simulink subsystem "Main_Controller_Scopes"  (R2025a)
settings: Solver=VariableStepAuto  StartTime=0.0  StopTime=10.0  RelTol=1e-3
Description:
  | Copyright 2025 The MathWorks, Inc.
settings Model: Creator=smiller  LastModifiedBy=smiller

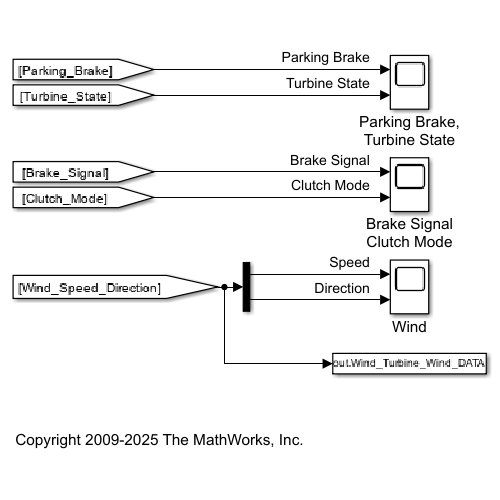
[thumbnail: Simulink's stored preview of the top-level diagram]
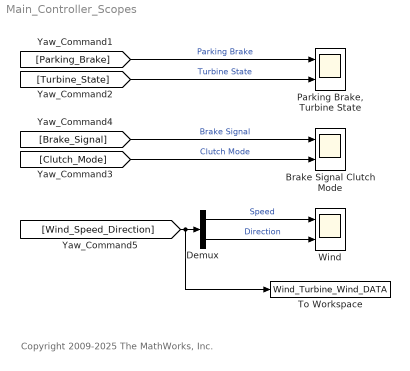
== system Main_Controller_Scopes ==
  note: Copyright 2009-2025 The MathWorks, Inc.
  Brake Signal Clutch Mode : Scope  NumInputPorts=2
      settings: TimeSpan=80  ActiveDisplayYMinimum=-1  ActiveDisplayYMaximum=1
  Demux : Demux  Outputs=2
  "Parking Brake, Turbine State" : Scope  NumInputPorts=2
      settings: TimeSpan=80  ActiveDisplayYMinimum=0  ActiveDisplayYMaximum=1  DataLoggingVariableName=ScopeData2
  To Workspace : ToWorkspace  VariableName=Wind_Turbine_Wind_DATA  SaveFormat=Structure With Time  SampleTime=-1
  Wind : Scope  NumInputPorts=2
      settings: TimeSpan=80  ActiveDisplayYMinimum=0  ActiveDisplayYMaximum=20  DataLoggingVariableName=Wind_Turbine_Wind_DATA
  wires:
  Demux/2 -> Wind/2  "Direction"
  [Clutch_Mode] -> Brake Signal Clutch Mode/2  "Clutch Mode"
  [Wind_Speed_Direction] -> Demux/1, To Workspace/1
  Demux/1 -> Wind/1  "Speed"
  [Parking_Brake] -> "Parking Brake, Turbine State"/1  "Parking Brake"
  [Turbine_State] -> "Parking Brake, Turbine State"/2  "Turbine State"
  [Brake_Signal] -> Brake Signal Clutch Mode/1  "Brake Signal"
